simulink model "DP_MotionRAO"  (R2022a)
settings: Solver=ode4  StartTime=0.0  StopTime=200  FixedStep=0.05  RelTol=1e-3  EnableMultiTasking=on
undefined symbols (not defined in the file): Hoerner, slcm, vessel
libraries: mssSimulink x6, simulink_extras x6
settings Model: Creator=Thor  LastModifiedBy=thor
settings SolverCC: AlgebraicLoopSolver=TrustRegion
settings DataIOCC: LimitDataPoints=on  SaveFormat=Array  SignalLoggingSaveFormat=ModelDataLogs  ReturnWorkspaceOutputs=off
settings OptimizationCC: ExpressionDepthLimit=2147483647  InitFltsAndDblsToZero=on  LifeSpan=inf
settings DebuggingCC: SaveWithParameterizedLinksMsg=none  UnderspecifiedInitializationDetection=Classic  MergeDetectMultiDrivingBlocksExec=none  SignalResolutionControl=TryResolveAllWithWarning  SolverPrmCheckMsg=warning  MultiTaskDSMMsg=warning  MultiTaskCondExecSysMsg=none  FcnCallInpInsideContextMsg=warning  UnconnectedInputMsg=warning  UnconnectedOutputMsg=warning  UnconnectedLineMsg=warning  StateNameClashWarn=warning  SFUnexpectedBacktrackingDiag=warning  SFNoUnconditionalDefaultTransitionDiag=warning  SFExecutionAtInitializationDiag=none  SFMachineParentedDataDiag=warning  ArithmeticOperatorsInVariantConditions=warning
settings HardwareCC: ProdBitPerPointer=32  ProdBitPerSizeT=32  ProdBitPerPtrDiffT=32  ProdLargestAtomicFloat=None  ProdIntDivRoundTo=Undefined  ProdEndianess=Unspecified  ProdWordSize=32  ProdHWDeviceType=32-bit Generic
settings ModelReferenceCC: PropagateSignalLabelsOutOfModel=off
settings SFSimCC: SimUseLocalCustomCode=off  CustomCodeUndefinedFunction=UseInterfaceOnly
settings RTWCC: RTWUseLocalCustomCode=off  DLArmComputeVersion=19.05
settings CodeAppCC: StateflowObjectComments=on
settings GRTTargetCC: TargetFcnLib=ansi_tfl_tmw.mat  TargetLangStandard=C89/C90 (ANSI)  CombineOutputUpdateFcns=off  GRTInterface=on
settings ConfigComp: CovMetricSettings=dw  CovSaveCumulativeToWorkspaceVar=on  CovSaveSingleToWorkspaceVar=on  CovExternalEMLEnable=off

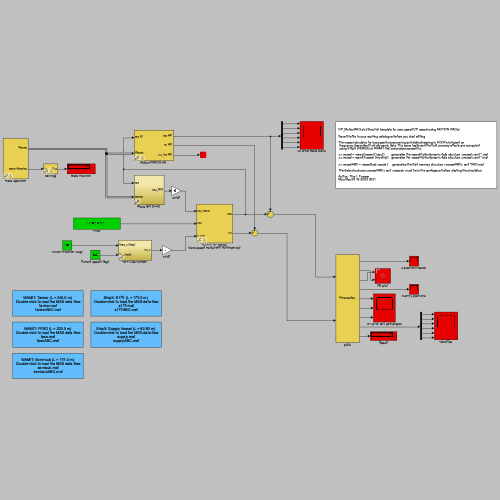
[thumbnail: Simulink's stored preview of the top-level diagram]
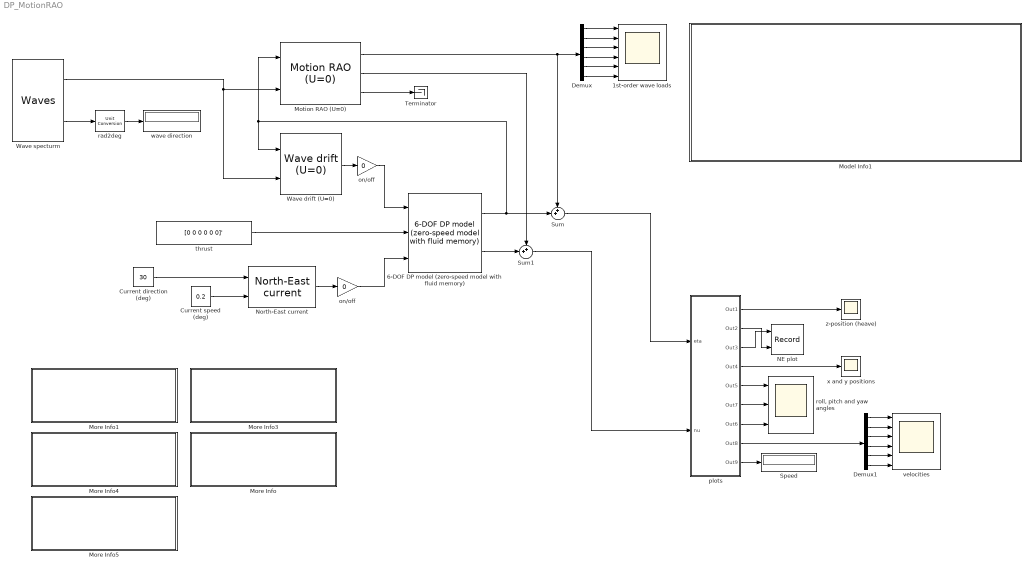
== system DP_MotionRAO ==
  "1st-order wave loads " : Scope  NumInputPorts=6
  "6-DOF DP model (zero-speed model with fluid memory) " : mssSimulink/Hydrodynamics/6-DOF DP model  (zero-speed model with fluid memory)  ABC=vesselABC  rho=1025  Axc=0.9*vessel.main.T*vessel.main.B  Ayc=0.9*vessel.main.T*vessel.main.Lpp  CX=1  CY_2D=Hoerner(vessel.main.B,vessel.main.T)
  Current direction (deg) : Constant  Value=30
  Current speed (deg) : Constant  Value=0.2
  Demux : Demux  Outputs=6
      settings: DisplayOption=none
  Demux1 : Demux  Outputs=6
      settings: DisplayOption=none
  Model Info1 : Subsystem  LoadFcn=slcm LoadBlock;  InitFcn=slcm('UpdateAllCMBlocksInThisModelInit')  mask(CMBlock){InitialSaveTempField=, InitialBlockCM=None, BlockCM=None, Frame=on, SaveTempField=, DisplayStringWithTags=|, MaskDisplayString=DP_MotionRAO.slx (Simulink template for zero-speed DP vessel using MOTION RAOs)\n\nSave this file to your working catalogue before you start editing\n\nThe vessel simulator for low-speed maneuvering and stationkeeping in 6 DOFs is based on\n frequency-dependent hydrodynamic data. The wave loads and the fluid-memory effects are computed\n using ShipX (VERES) or WAMIT that are postprocessed by:\n\n>> vessel = veres2vessel ('input')        generates the vessel/hydrodynamic data structure <vessel> and *.mat \n>> vessel = wamit2vessel ('myship'')   generates the vessel/hydrodynamic data structure <vessel> and *.mat \n\n>> vesselABC = vessel2ss( vessel )     generates the fluid memory structure <vesselABC> and *ABC.mat\n\nThe data structures <vesselABC> and <vessel> must be in the workspace before starting the simulation.\n\nAuthor: Thor I. Fossen\nMon Mar 29 19:20:52 2021, HorizontalTextAlignment=Left, LeftAlignmentValue=0.02, SourceBlockDiagram=DP_MotionRAO, TagMaxNumber=20, CMTag1=, CMTag2=, CMTag3=, CMTag4=, CMTag5=, CMTag6=, CMTag7=, CMTag8=, CMTag9=, CMTag10=, CMTag11=, CMTag12=, CMTag13=, CMTag14=, CMTag15=, CMTag16=, CMTag17=, CMTag18=, CMTag19=, CMTag20=}
      mask DisplayStringWithTags=|
      | DP_MotionRAO.slx (Simulink template for zero-speed DP vessel using MOTION RAOs)\n
      | Save this file to your working catalogue before you start editing\n
      | The vessel simulator for low-speed maneuvering and stationkeeping in 6 DOFs is based on\n frequency-dependent hydrodynamic data. The wave loads and the fluid-memory effects are computed\n using ShipX (VERES) or WAMIT that are postprocessed by:\n
      | >> vessel = veres2vessel ('input')        generates the vessel/hydrodynamic data structure <vessel> and *.mat
      | >> vessel = wamit2vessel ('myship'')   generates the vessel/hydrodynamic data structure <vessel> and *.mat
      |
      | >> vesselABC = vessel2ss( vessel )     generates the fluid memory structure <vesselABC> and *ABC.mat
      |
      | The data structures <vesselABC> and <vessel> must be in the workspace before starting the simulation.
      |
      | Author: Thor I. Fossen
      | %<LastModificationDate>
      mask help: This block allows revision control information to be displayed within the model.
      settings: CopyFcn=slcm CopyBlock;  DeleteFcn=slcm Cancel;  PostSaveFcn=slcm('UpdateAllCMBlocksInThisModel')  NameChangeFcn=slcm Rename;  OpenFcn=slcm
      mask Display: text(str2num(LeftAlignmentValue), 0.5, MaskDisplayString, 'HorizontalAlignment', HorizontalTextAlignment)
  More Info : Subsystem
      settings: OpenFcn=load('supply'),load('supplyABC');disp('MSS supply vessel data set (L = 82.80 m) loaded')
      mask Display: disp('ShipX: Supply Vessel (L = 82.80 m)\n  Double-click to load the MSS data files:\n supply.mat\n supplyABC.mat')
  More Info1 : Subsystem
      settings: OpenFcn=load('tanker'),load('tankerABC');disp('MSS tanker data set (L = 246.0 m) loaded')
      mask Display: disp('WAMIT: Tanker (L = 246.0 m)\n  Double-click to load the MSS data files:\n tanker.mat\n tankerABC.mat')
  More Info3 : Subsystem
      settings: OpenFcn=load('s175'),load('s175ABC');disp('MSS S175 data set (L = 175.0 m) loaded')
      mask Display: disp('ShipX: S175 (L = 175.0 m)\n  Double-click to load the MSS data files:\n s175.mat\n s175ABC.mat')
  More Info4 : Subsystem
      settings: OpenFcn=load('fpso'),load('fpsoABC');disp('MSS FPSO data set (L = 200.0 m) loaded')
      mask Display: disp('WAMIT: FPSO (L = 200.0 m)\n  Double-click to load the MSS data files:\n fpso.mat\n fpsoABC.mat')
  More Info5 : Subsystem
      settings: OpenFcn=load('semisub'),load('semisubABC');disp('MSS semi-sub data set (L = 115.0 m) loaded')
      mask Display: disp('WAMIT: Semi-sub (L = 115.0 m)\n  Double-click to load the MSS data files:\n semisub.mat\n semisubABC.mat')
  "Motion RAO (U=0) " : mssSimulink/Hydrodynamics/Motion RAO (U=0)  RAO_Freq=vessel.motionRAO.w  RAO_Dir=vessel.headings  RAO_Vel=vessel.velocities  RAO_Amp=vessel.motionRAO.amp  RAO_Phase=vessel.motionRAO.phase  RAO_add_omega_0=on  RAO_add_omega_inf=on  RAO_yaw_quantization_flag=on  RAO_yaw_quant=5*pi/180  RAO_yaw_back=1.2*pi/180  RAO_speed_backlash_flag=on  RAO_speed_back=2  RAO_smoothing_flag=on
  NE plot : Record  FileSettingsInternal="{\"entries\":[{\"content\":{\"excelSettings\":{\"content\":{},\"type\":\"Streamout.ExcelSettings\"}},\"type\":\"Streamout.FileSettingStorage\",\"uuid\":\"8ec5b344-6cd9-46fc-82cc-06c2a8d6b921\"}],\"packageUris\":[\"http://schema.mathworks.com/mf0/streamout_blocks/R2020a\"],\"version\":\"1.0\"}"  Layout=[1 1]  SignalsInternal="{\"entries\":[{\"content\":{\"signals\":[{\"content\":{\"blockPath\":[\"DP_MotionRAO/NE plot\"],\"channel\":[],\"dimensions\":[1],\"domain\":\"DP_MotionRAO/NE plot\",\"lineColor\":\"#a2142f\",\"plots\":[1],\"port\":1,\"sid\":[\"\"],\"signalID\":1179,\"signalName\":\"plots:3\"},\"type\":\"RecordBlkView.Signal\",\"uuid\":\"bf50ee90-d15c-4815-9bf9-50b91a0ff69b\"},{\"content\":{\"blockPath\":[\"DP_MotionRAO/NE plot\"],\"channel\":[],\"dimensions\":[1],\"domain\":\"DP_MotionRAO/NE plot\",\"lineColor\":\"#139fff\",\"plots\":[1],\"port\":2,\"sid\":[\"\"],\"signalID\":1183,\"signalName\":\"plots:2\"},\"type\":\"RecordBlkView.Signal\",\"uuid\":\"167ec1d4-da96-423a-9d15-31afaff2b47b\"}]},\"type\":\"RecordBlkView.InputSignals\",\"uuid\":\"9370312c-4758-4aab-aeed-be48e91296cf\"}],\"packageUris\":[\"http://schema.mathworks.com/mf0/streamout_blocks/R2020a\"],\"version\":\"1.0\"}"  VisualizationBindings="{\"xyplotplugin\":{\"info\":[{\"series\":[{\"bindingParametersList\":[{\"parameter\":\"X-Axis\",\"signalID\":1179,\"signalName\":\"plots:3\"},{\"parameter\":\"Y-Axis\",\"signalID\":1183,\"signalName\":\"plots:2\"}],\"seriesID\":26157}],\"subplotID\":1}]}}"  CompatibilityTag=XY  st=-1
  "North-East current " : mssSimulink/Environment/Current/North-East current  SystemSampleTime=-1  VariantActivationTime=update diagram  Latency=0  AutoFrameSizeCalculation=off
  Speed : Display
  Sum : Sum  Inputs=++|
  Sum1 : Sum  Inputs=++|
  Terminator : Terminator
  "Wave drift (U=0) " : mssSimulink/Hydrodynamics/Wave drift (U=0)  SystemSampleTime=-1  VariantActivationTime=update diagram  Latency=0  AutoFrameSizeCalculation=off
  Wave specturm : mssSimulink/Environment/Waves/Waves  spectrum_type=ITTC  disp_flag=off  plot_spectrum=off  plot_realization=off  hs=5  omega_peak=-1  psi_mean=30/(180/pi)  gamma=-1  spread=2  depth=inf  nfreq=20  ndir=10  energylim=0.005  freq_cutoff=3  dir_cutoff=0  rand_seed=0  rand_freq=on  rand_dir=on  Zeta_a=0  Omega=0  Phase=0  Wavenum=0  Psi=0
  on/off : Gain  Gain=0
  "on/off " : Gain  Gain=0
  plots : Subsystem
      mask Display: disp('time-series')
  rad2deg : mssSimulink/Utilities/Math Operations/Unit Conversion  in=rad2deg
  "roll, pitch and yaw angles" : Scope  NumInputPorts=3
  thrust : Constant  Value=[0 0 0 0 0 0]'
  velocities : Scope  NumInputPorts=6
  wave direction : Display
  x and y positions : Scope
  z-position (heave) : Scope
  wires:
  thrust/1 -> "6-DOF DP model (zero-speed model with fluid memory) "/2
  "6-DOF DP model (zero-speed model with fluid memory) "/1 -> "Motion RAO (U=0) "/1, "Wave drift (U=0) "/1, Sum/2
  Demux/1 -> "1st-order wave loads "/1
  Demux/2 -> "1st-order wave loads "/2
  Demux/3 -> "1st-order wave loads "/3
  Demux/4 -> "1st-order wave loads "/4
  Demux/5 -> "1st-order wave loads "/5
  Demux/6 -> "1st-order wave loads "/6
  Wave specturm/1 -> "Motion RAO (U=0) "/2, "Wave drift (U=0) "/2
  Wave specturm/2 -> rad2deg/1
  rad2deg/1 -> wave direction/1
  "Motion RAO (U=0) "/1 -> Demux/1, Sum/1
  "Motion RAO (U=0) "/2 -> Sum1/1
  "Motion RAO (U=0) "/3 -> Terminator/1
  "North-East current "/1 -> "on/off "/1
  "on/off "/1 -> "6-DOF DP model (zero-speed model with fluid memory) "/3
  Current speed (deg)/1 -> "North-East current "/2
  Current direction (deg)/1 -> "North-East current "/1
  plots/3(Out3) -> NE plot/1
  plots/2(Out2) -> NE plot/2
  plots/4(Out4) -> x and y positions/1
  plots/5(Out5) -> "roll, pitch and yaw angles"/1
  plots/6(Out7) -> "roll, pitch and yaw angles"/2
  plots/7(Out6) -> "roll, pitch and yaw angles"/3
  plots/1(Out1) -> z-position (heave)/1
  Demux1/1 -> velocities/1
  Demux1/2 -> velocities/2
  Demux1/3 -> velocities/3
  Demux1/4 -> velocities/4
  Demux1/5 -> velocities/5
  Demux1/6 -> velocities/6
  Sum1/1 -> plots/2(nu)
  plots/8(Out8) -> Demux1/1
  plots/9(Out9) -> Speed/1
  Sum/1 -> plots/1(eta)
  on/off/1 -> "6-DOF DP model (zero-speed model with fluid memory) "/1
  "Wave drift (U=0) "/1 -> on/off/1
  "6-DOF DP model (zero-speed model with fluid memory) "/2 -> Sum1/2

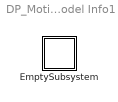
== system DP_MotionRAO/Model Info1 ==
  EmptySubsystem : Subsystem

== system DP_MotionRAO/More Info ==

== system DP_MotionRAO/More Info1 ==

== system DP_MotionRAO/More Info3 ==

== system DP_MotionRAO/More Info4 ==

== system DP_MotionRAO/More Info5 ==

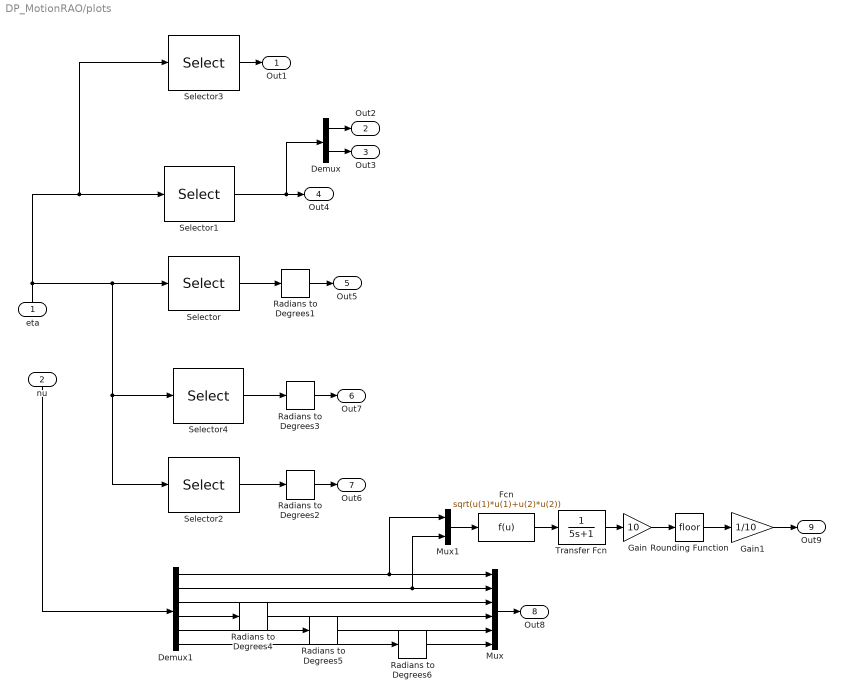
== system DP_MotionRAO/plots ==
  eta : Inport
  nu : Inport  Port=2
  Demux : Demux  Outputs=2
      settings: DisplayOption=none
  Demux1 : Demux  Outputs=6
      settings: DisplayOption=none
  Fcn : Fcn  Expr=sqrt(u(1)*u(1)+u(2)*u(2))
  Gain : Gain  Gain=10
  Gain1 : Gain  Gain=1/10
  Mux : Mux  Inputs=6
  Mux1 : Mux  Inputs=2
  Radians to Degrees{1..6} (6 alike) : simulink_extras/Transformations/Radians to Degrees
  Rounding Function : Rounding
  Selector : Selector  InputPortWidth=6  IndexOptions=Index vector (dialog)  Indices=[4 ]  OutputSizes=1
  Selector1 : Selector  InputPortWidth=6  IndexOptions=Index vector (dialog)  Indices=[1 2]  OutputSizes=1
  Selector2 : Selector  InputPortWidth=6  IndexOptions=Index vector (dialog)  Indices=[6]  OutputSizes=1
  Selector3 : Selector  InputPortWidth=6  IndexOptions=Index vector (dialog)  Indices=[3]  OutputSizes=1
  Selector4 : Selector  InputPortWidth=6  IndexOptions=Index vector (dialog)  Indices=[5]  OutputSizes=1
  Transfer Fcn : TransferFcn  Denominator=[5 1]
  Out1 : Outport
  Out2 : Outport  Port=2
  Out3 : Outport  Port=3
  Out4 : Outport  Port=4
  Out5 : Outport  Port=5
  Out7 : Outport  Port=6
  Out6 : Outport  Port=7
  Out8 : Outport  Port=8
  Out9 : Outport  Port=9
  wires:
  eta/1 -> Selector3/1, Selector1/1, Selector/1, Selector2/1, Selector4/1
  Selector/1 -> Radians to Degrees1/1
  Selector1/1 -> Demux/1, Out4/1
  Selector2/1 -> Radians to Degrees2/1
  Selector3/1 -> Out1/1
  Demux/1 -> Out2/1
  Demux/2 -> Out3/1
  Radians to Degrees1/1 -> Out5/1
  Radians to Degrees2/1 -> Out6/1
  Selector4/1 -> Radians to Degrees3/1
  Radians to Degrees3/1 -> Out7/1
  nu/1 -> Demux1/1
  Demux1/1 -> Mux/1, Mux1/1
  Demux1/2 -> Mux/2, Mux1/2
  Demux1/3 -> Mux/3
  Demux1/4 -> Radians to Degrees4/1
  Demux1/5 -> Radians to Degrees5/1
  Demux1/6 -> Radians to Degrees6/1
  Radians to Degrees6/1 -> Mux/6
  Radians to Degrees5/1 -> Mux/5
  Radians to Degrees4/1 -> Mux/4
  Mux/1 -> Out8/1
  Fcn/1 -> Transfer Fcn/1
  Mux1/1 -> Fcn/1
  Rounding Function/1 -> Gain1/1
  Gain/1 -> Rounding Function/1
  Gain1/1 -> Out9/1
  Transfer Fcn/1 -> Gain/1

== system DP_MotionRAO/Model Info1/EmptySubsystem ==
